simulink model "case_10_fast_to_slow_start_close"  (R2025b)
settings: Solver=VariableStepAuto  StartTime=0.0  StopTime=120  RelTol=1e-3
settings Model: Creator=sanborkl  LastModifiedBy=sanborkl
settings DebuggingCC: UnderSpecifiedDimensionMsg=warning

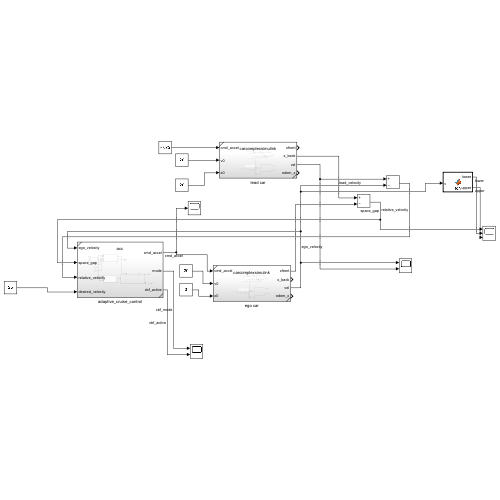
[thumbnail: Simulink's stored preview of the top-level diagram]
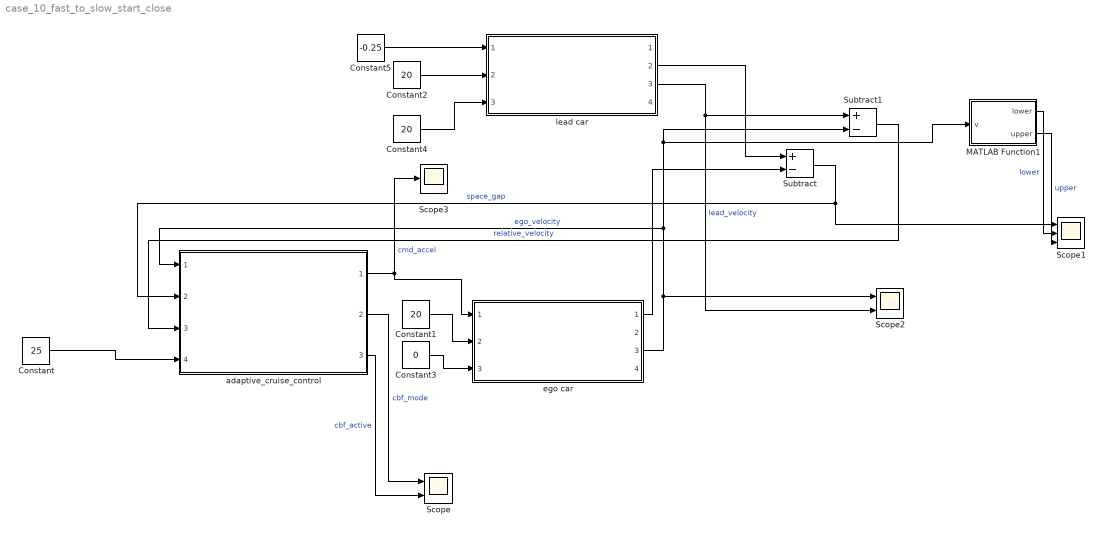
== system case_10_fast_to_slow_start_close ==
  Constant : Constant  Value=25
  Constant1 : Constant  Value=20
  Constant2 : Constant  Value=20
  Constant3 : Constant  Value=0
  Constant4 : Constant  Value=20
  Constant5 : Constant  Value=-0.25
  MATLAB Function1 : MATLAB Function  TreatAsAtomicUnit=on
  Scope : Scope  NumInputPorts=2
      settings: ActiveDisplayYMinimum=-0.24999999999999994  ActiveDisplayYMaximum=2.25
  Scope1 : Scope  NumInputPorts=3
      settings: ActiveDisplayYMinimum=-1.2359711495869279  ActiveDisplayYMaximum=61.248441238842993  YLabel=m
  Scope2 : Scope  NumInputPorts=2
      settings: ActiveDisplayYMinimum=-2.4999999999999996  ActiveDisplayYMaximum=22.5  YLabel=m/s  DataLoggingVariableName=ScopeData2
  Scope3 : Scope
      settings: ActiveDisplayYMinimum=-2.2406945872866526  ActiveDisplayYMaximum=0.52747473676168044  YLabel=m/s^2  DataLoggingVariableName=ScopeData3
  Subtract : Sum  Inputs=+-
  Subtract1 : Sum  Inputs=+-
  adaptive_cruise_control : Subsystem  ReferencedSubsystem=acc
  ego car : Subsystem  ReferencedSubsystem=carcomplexsimulink
  lead car : Subsystem  ReferencedSubsystem=carcomplexsimulink
  wires:
  adaptive_cruise_control/1 -> ego car/1, Scope3/1  "cmd_accel"
  ego car/3 -> Subtract1/2, MATLAB Function1/1(v), adaptive_cruise_control/1, Scope2/1  "ego_velocity"
  lead car/2 -> Subtract/1
  ego car/1 -> Subtract/2
  Subtract/1 -> Scope1/1, adaptive_cruise_control/2  "space_gap"
  lead car/3 -> Scope2/2, Subtract1/1  "lead_velocity"
  Subtract1/1 -> adaptive_cruise_control/3  "relative_velocity"
  Constant/1 -> adaptive_cruise_control/4
  adaptive_cruise_control/2 -> Scope/1  "cbf_mode"
  Constant1/1 -> ego car/2
  Constant2/1 -> lead car/2
  Constant3/1 -> ego car/3
  Constant4/1 -> lead car/3
  Constant5/1 -> lead car/1
  adaptive_cruise_control/3 -> Scope/2  "cbf_active"
  MATLAB Function1/1(lower) -> Scope1/2  "lower"
  MATLAB Function1/2(upper) -> Scope1/3  "upper"

== matlab function case_10_fast_to_slow_start_close/MATLAB Function1 ==
  data: v input; lower output; upper output
function [lower, upper] = fcn(v)

lower = 2 * v + 5;
upper = 2 * v + 15;
